simulink model "BlocoHidraulicoLAC_closeLoop"  (R2026a)
settings: Solver=ode15s  StopTime=5  FixedStep=0.001  MaxStep=1e-4
values from neighbouring files (symbols this model uses):
  Gamma = sys_d.B    [sintese_lqi_luenberger_lac.m]    (also in sintese_lqi_luenberger_lac_bateria_de_ensaio.m)
  K_i = -K_aug(3)    [sintese_lqi_luenberger_lac.m]    (also in sintese_lqi_luenberger_lac_bateria_de_ensaio.m)
  K_lqr = [K_pos, K_vel]    [sintese_lqi_luenberger_lac.m]    (also in sintese_lqi_luenberger_lac_bateria_de_ensaio.m)
  L_obs = place(Phi', Cx', polos_obs)'    [sintese_lqi_luenberger_lac.m]    (also in sintese_lqi_luenberger_lac_bateria_de_ensaio.m)
  Phi = sys_d.A    [sintese_lqi_luenberger_lac.m]    (also in sintese_lqi_luenberger_lac_bateria_de_ensaio.m)
undefined symbols (not defined in the file or in its folder): sigbuilder_block
(part 2 of 4)

== matlab function BlocoHidraulicoLAC_closeLoop/MATLAB Function ==
  settings: updateMethod=DISCRETE
  data: x_ref_mm input; duty_cycle_lac output; x_med_mm input; Phi input; Gamma input; K_lqr input; K_i input; L_obs input; dt input; x_est_mm output; v_est_mms output
function [duty_cycle_lac, x_est_mm, v_est_mms] = ...
    ecu_controle_posicao_lac_lqi(x_ref_mm, x_med_mm, Phi, Gamma, K_lqr, K_i, L_obs, dt)
%#codegen
% =========================================================================
% ECU AUTOMOTIVA: CONTROLE DE POSIÇÃO DO LAC VIA LQI + LUENBERGER
% Equivalente funcional do firmware em linguagem C (AURIX TC375)
% =========================================================================
% Entradas:
%   x_ref_mm       : Referência de deslocamento linear do êmbolo [mm]
%   x_med_mm       : Deslocamento medido pelo sensor/encoder da planta [mm]
%   Phi            : Matriz de estados do modelo discreto (2x2)
%   Gamma          : Vetor de entrada do modelo discreto (2x1)
%   K_lqr          : Ganhos dos estados proporcionais [K_pos, K_vel] (1x2)
%   K_i            : Ganho da ação integral de posição (escalar)
%   L_obs          : Vetor de ganhos do Observador de Luenberger (2x1)
%   dt             : Passo de amostragem numérico da ECU [s]
%
% Saídas:
%   duty_cycle_lac : Comando PWM de acionamento do motor [-100% a +100%]
%   x_est_mm       : Posição estimada pelo observador [mm]
%   v_est_mms      : Velocidade estimada pelo observador [mm/s]
% =========================================================================

%% 1. LIMITES MECÂNICOS DO ATUADOR FÍSICO
X_MIN_MM = 0.0;    % Batente mecânico traseiro (repouso) [mm]
X_MAX_MM = 53.7;   % Batente mecânico dianteiro (curso total) [mm]

%% 2. MEMÓRIA INTERNA DE ESTADOS (PERSISTENT / ESTÁTICAS DE FIRMWARE)
persistent xhat vhat integral_pos last_u
if isempty(xhat)
    xhat         = 0.0; % Posição estimada [mm]
    vhat         = 0.0; % Velocidade estimada [mm/s]
    integral_pos = 0.0; % Acumulador integral do erro [mm*s]
    last_u       = 0.0; % Último comando PWM efetivamente aplicado [-100 a +100]
end

%% 3. CONDICIONAMENTO DA REFERÊNCIA
% Garante que a referência nunca demande posição além dos fins de curso
x_ref_clamped = max(X_MIN_MM, min(X_MAX_MM, double(x_ref_mm)));
pos_real      = double(x_med_mm);

%% 4. OBSERVADOR DE LUENBERGER DISCRETO (PREDITOR-CORRETOR)
% Cálculo da inovação (erro de observação da saída de posição)
innov = pos_real - xhat;

% Atualização temporal dos estados estimados
xhat_new = Phi(1,1)*xhat + Phi(1,2)*vhat + Gamma(1)*last_u + L_obs(1)*innov;
vhat_new = Phi(2,1)*xhat + Phi(2,2)*vhat + Gamma(2)*last_u + L_obs(2)*innov;

xhat = xhat_new;
vhat = vhat_new;

%% 5. LEI DE CONTROLE LQI DE POSIÇÃO
erro_pos = x_ref_clamped - xhat;

% Candidato à integração do erro
integral_cand = integral_pos + erro_pos * dt;

% Lei de controle ótima não saturada
u_unclamped = (K_lqr(1) * erro_pos) - (K_lqr(2) * vhat) + (K_i * integral_cand);

%% 6. ANTI-WINDUP CONDICIONAL IDÊNTICO AO FIRMWARE AURIX
% Clamping rígido da ação integral quando satura na mesma direção do esforço
if (u_unclamped > 100.0 && erro_pos > 0.0)
    u_cmd = 100.0;
    % Congela a integração (não atualiza integral_pos)
elseif (u_unclamped < -100.0 && erro_pos < 0.0)
    u_cmd = -100.0;
    % Congela a integração (não atualiza integral_pos)
else
    integral_pos = integral_cand;
    u_cmd = u_unclamped;
    if u_cmd > 100.0
        u_cmd = 100.0;
    elseif u_cmd < -100.0
        u_cmd = -100.0;
    end
end

%% 7. ATUALIZAÇÃO DAS SAÍDAS E REGISTRADOR DE RETORNO
duty_cycle_lac = u_cmd;
last_u         = u_cmd;

x_est_mm  = xhat;
v_est_mms = vhat;

end
% function [duty_cycle_lac, u_mcv, u_pfv, u_irl, u_orl, x_est_mm, v_est_mms] = ...
%     ecu_controle_posicao_lac_lqi(x_ref_mm, x_med_mm, hab_adas, Phi, Gamma, K_lqr, K_i, L_obs, dt)
% %#codegen
% % =========================================================================
% % ECU AUTOMOTIVA: CONTROLE DE POSIÇÃO DO ATUADOR LINEAR (LAC) VIA LQI
% % =========================================================================
% % Entradas:
% %   x_ref_mm       : Posição de referência do êmbolo [mm]
% %   x_med_mm       : Posição medida pelo sensor/encoder da planta [mm]
% %   hab_adas       : Habilitação da função autônoma (1 = Ativo, 0 = Standby)
% %   Phi            : Matriz do modelo discreto (2x2) [pos; vel]
% %   Gamma          : Vetor de entrada do modelo discreto (2x1)
% %   K_lqr          : Vetor de ganhos dos estados [K_pos, K_vel] (1x2)
% %   K_i            : Ganho da ação integral de posição (escalar)
% %   L_obs          : Ganhos do Observador de Luenberger (2x1) [L_pos; L_vel]
% %   dt             : Período de amostragem do controle [s]
% %
% % Saídas:
% %   duty_cycle_lac : Sinal PWM para a ponte H do motor [-100% a +100%]
% %   u_mcv          : Válvula de corte mestre (NA: 1 = Energizada/Fechada)
% %   u_pfv          : Válvula de alimentação (NF: 1 = Energizada/Aberta)
% %   u_irl          : Válvula de entrada do caliper (NA: 0 = Aberta)
% %   u_orl          : Válvula de descarga/retorno (NF: 0 = Fechada)
% %   x_est_mm       : Posição estimada pelo observador [mm]
% %   v_est_mms      : Velocidade estimada pelo observador [mm/s]
% % =========================================================================
% 
% %% 1. LIMITES OPERACIONAIS E FÍSICOS
% X_MAX_MM = 53.7;  % Fim de curso mecânico máximo do êmbolo [mm]
% X_MIN_MM = 0.0;   % Posição de repouso mecânico do êmbolo [mm]
% 
% %% 2. MEMÓRIA INTERNA DE ESTADOS (PERSISTENT)
% persistent xhat vhat z_int u_ant
% if isempty(xhat)
%     xhat  = 0.0;  % Posição estimada [mm]
%     vhat  = 0.0;  % Velocidade estimada [mm/s]
%     z_int = 0.0;  % Integrador do erro de posição [mm*s]
%     u_ant = 0.0;  % Comando PWM anterior aplicado [-100 a +100]
% end
% 
% %% 3. CONDICIONAMENTO DAS ENTRADAS E REFERÊNCIAS
% % Saturação da referência de posição dentro dos batentes físicos
% x_ref_sat = max(X_MIN_MM, min(X_MAX_MM, double(x_ref_mm)));
% y_med     = double(x_med_mm);
% 
% %% 4. OBSERVADOR DE LUENBERGER DISCRETO (PREDITOR-CORRETOR)
% % Inovação baseada na leitura do sensor de posição físico
% innov = y_med - xhat;
% 
% % Predição e correção temporal de estados com as matrizes externas
% xhat_next = Phi(1,1)*xhat + Phi(1,2)*vhat + Gamma(1)*u_ant + L_obs(1)*innov;
% vhat_next = Phi(2,1)*xhat + Phi(2,2)*vhat + Gamma(2)*u_ant + L_obs(2)*innov;
% 
% % Atualização dos estados estimados
% xhat = xhat_next;
% vhat = vhat_next;
% 
% %% 5. GESTÃO OPERACIONAL DAS VÁLVULAS SOLENOIDES (MODO ADAS)
% if hab_adas > 0.5
%     % --- MODO ATIVO DE FRENAGEM (ACC / AEB) ---
%     % MCV fechada (isola pedal), PFV aberta (conecta LAC ao circuito)
%     % IRL aberta (livre fluxo para a pinça), ORL fechada (sem alívio ao dreno)
%     u_mcv = 1.0;
%     u_pfv = 1.0;
%     u_irl = 0.0; 
%     u_orl = 0.0;
% 
%     %% 6. LEI DE CONTROLE LQI DE POSIÇÃO
%     erro_pos = x_ref_sat - xhat;
% 
%     % Candidato à atualização integral
%     z_cand = z_int + erro_pos * dt;
% 
%     % Lei de controle LQI: u = -Kx*xhat + Ki*z
%     % u_lqi = K_lqr(1)*(x_ref - xhat) - K_lqr(2)*vhat + K_i*z
%     u_unclamped = (K_lqr(1) * erro_pos) - (K_lqr(2) * vhat) + (K_i * z_cand);
% 
%     % Saturação do atuador motor [-100% a +100%]
%     u_sat = max(-100.0, min(100.0, u_unclamped));
% 
%     % Anti-windup condicional por integração clamped
%     is_saturated = (u_sat ~= u_unclamped);
%     if is_saturated
%         % Congela o integrador se a saturação estiver na mesma direção do erro
%         if (u_sat >= 100.0 && erro_pos > 0.0) || (u_sat <= -100.0 && erro_pos < 0.0)
%             % Mantém z_int anterior (não integra)
%         else
%             z_int = z_cand;
%         end
%     else
%         z_int = z_cand;
%     end
% 
%     duty_cycle_lac = u_sat;
% 
% else
%     % --- MODO STANDBY / REPOUSO ---
%     % Circuito hidráulico despressurizado e conectado ao pedal/reservatório
%     u_mcv = 0.0; % Aberta
%     u_pfv = 0.0; % Fechada
%     u_irl = 0.0; % Aberta
%     u_orl = 0.0; % Fechada
% 
%     duty_cycle_lac = 0.0;
%     z_int = 0.0; % Zera integrador
% end
% 
% %% 7. ATUALIZAÇÃO DE REGISTRADORES E SAÍDAS DO BLOCO
% u_ant = duty_cycle_lac;
% 
% x_est_mm  = xhat;
% v_est_mms = vhat;
% 
% end
% 
% 
% 
% 
% % function [duty_cycle_ecu, u_mcv, u_pfv, u_irl, u_orl] = ecu_control_valves_fcn(P_roda_pa, P_ref_pa, K_est, K_i, L_obs, dt)
% % %#codegen
% % % =========================================================================
% % % ECU AUTOMOTIVA: CONTROLE INDIRETO DE PRESSÃO VIA POSIÇÃO DO LAC
% % % =========================================================================
% % % Entradas:
% % %   P_roda_pa  : Leitura do sensor de pressão no caliper [Pa]
% % %   P_ref_pa   : Referência de pressão enviada pelo piloto/sistema [Pa]
% % %   K_est      : Ganhos do LQI para estados [x, x_dot, P] (1x3)
% % %   K_i        : Ganho integral do LQI de posição (escalar)
% % %   L_obs      : Ganhos do Observador de Luenberger [L_vel; L_pres] (2x1)
% % %   dt         : Período de amostragem da ECU [s]
% % %
% % % Saídas:
% % %   duty_cycle_ecu : Comando PWM para a ponte H do motor [-100% a +100%]
% % %   u_mcv, u_pfv, u_irl, u_orl : Sinais ON/OFF para os solenoides das válvulas
% % % =========================================================================
% % 
% % %% 1. PARÂMETROS FIXOS DE MATRIZES DA ECU
% % A_lac   = 2.85e-4;       % Área do êmbolo do LAC [m^2]
% % tau_m   = 0.140;         % Constante de tempo mecânica [s]
% % K_drv   = 0.085;         % Ganho de velocidade fuso [m/s]
% % C_eq    = 9.51e-12;      % Capacitância equivalente [m^3/Pa]
% % 
% % % Submatrizes do observador reduzido de ordem 2 [x_dot; p]
% % A_sub = [-1.0/tau_m, 0.0;
% %           A_lac/C_eq, 0.0];
% % B_sub = [K_drv/tau_m; 
% %          0.0];
% % 
% % % Banda morta hidráulica de histerese (~1.5 PSI) para evitar oscilação de válvulas
% % BANDA_MORTA_PA = 1.5 * 6894.757;
% % 
% % %% 2. MEMÓRIA INTERNA DE ESTADOS ESTIMADOS DA ECU (PERSISTENT)
% % persistent x_est x_dot_est p_est erro_int_pos u_sat_ant
% % if isempty(x_est)
% %     x_est        = 0.0;
% %     x_dot_est    = 0.0;
% %     p_est        = 0.0;
% %     erro_int_pos = 0.0;
% %     u_sat_ant    = 0.0;
% % end
% % 
% % %% 3. MAPEAMENTO INDIRETO: PRESSÃO DE REFERÊNCIA -> POSIÇÃO DO LAC
% % % Em regime permanente hidráulico: delta_V = A_lac * x = C_eq * P
% % x_ref = (C_eq / A_lac) * double(P_ref_pa);
% % x_ref = max(0.0, min(0.0537, x_ref)); % Saturação no curso físico do atuador
% % 
% % %% 4. OBSERVADOR DE LUENBERGER REDUZIDO (ESTIMAÇÃO DE VELOCIDADE E PRESSÃO)
% % erro_estimacao = double(P_roda_pa) - p_est;
% % 
% % % Derivadas estimadas realimentadas pelo erro do sensor de pressão + comando anterior aplicado
% % x_dot_dot_est = A_sub(1,1)*x_dot_est + L_obs(1)*erro_estimacao + B_sub(1)*u_sat_ant;
% % p_dot_est     = A_sub(2,1)*x_dot_est + L_obs(2)*erro_estimacao;
% % 
% % % Integração numérica de Euler dos estados estimados
% % x_dot_est = x_dot_est + x_dot_dot_est * dt;
% % p_est     = max(0.0, p_est + p_dot_est * dt);
% % x_est     = max(0.0, min(0.0537, x_est + x_dot_est * dt));
% % 
% % %% 5. LEI DE CONTROLE LQI INDIRETO FOCADO NA POSIÇÃO DO LAC
% % % Erro instantâneo de deslocamento mecânico do fuso
% % erro_pos = x_ref - x_est;
% % 
% % % Cálculo da ação de controle ótimo por realimentação de estados + ação integral
% % % u = K_pos * (x_ref - x) - K_vel * x_dot + Ki * erro_integral
% % u_controle = K_est(1) * erro_pos - K_est(2) * x_dot_est + double(K_i) * erro_int_pos;
% % 
% % % Saturação física unitária do motor (-1.0 a +1.0)
% % u_sat = max(-1.0, min(1.0, u_controle));
% % 
% % %% 6. MÁQUINA DE ESTADOS HÍBRIDA (GERENCIAMENTO DAS VÁLVULAS)
% % erro_pressao_pa = double(P_ref_pa) - double(P_roda_pa);
% % 
% % if erro_pressao_pa > BANDA_MORTA_PA
% %     %% --- MODO APPLY (Aumento Ativo de Pressão) ---
% %     % Circuito conectado do LAC para a roda; dreno fechado
% %     u_mcv = 1; u_pfv = 1; u_irl = 1; u_orl = 0;
% % 
% %     % Acúmulo do integrador com Anti-Windup rígido no curso em metros
% %     erro_int_pos = erro_int_pos + erro_pos * dt;
% %     if erro_int_pos > 0.020;  erro_int_pos = 0.020;  end  % Máx: 20 mm.s
% %     if erro_int_pos < -0.020; erro_int_pos = -0.020; end
% % 
% %     duty_cycle_ecu = u_sat * 100.0;
% % 
% % elseif erro_pressao_pa < -BANDA_MORTA_PA
% %     %% --- MODO RELEASE (Alívio Rápido de Pressão) ---
% %     % Drena fluido do caliper para o reservatório
% %     u_mcv = 0; u_pfv = 0; u_irl = 0; u_orl = 1;
% % 
% %     % Reseta a ação integral para evitar overshoot no retorno
% %     erro_int_pos = 0.0;
% % 
% %     % Recuo seguro do LAC: acompanha x_ref de volta à posição inicial
% %     if x_est > 0.001
% %         duty_cycle_ecu = min(0.0, max(-50.0, u_sat * 100.0));
% %     else
% %         duty_cycle_ecu = 0.0;
% %     end
% % 
% % else
% %     %% --- MODO HOLD (Retenção Hidráulica no Patamar) ---
% %     % Válvulas calam o caliper retendo a pressão; desliga o motor para poupar energia
% %     u_mcv = 1; u_pfv = 0; u_irl = 0; u_orl = 0;
% % 
% %     duty_cycle_ecu = 0.0;
% % end
% % 
% % % Limitação final de segurança da ponte H
% % duty_cycle_ecu = max(-100.0, min(100.0, duty_cycle_ecu));
% % 
% % % Atualiza o comando efetivo repassado para o observador no próximo passo
% % u_sat_ant = duty_cycle_ecu / 100.0;
% % 
% % end
% % 
% % % function [duty_cycle_ecu, u_mcv, u_pfv, u_irl, u_orl] = ecu_control_valves_fcn(P_roda_pa, P_ref_pa, K_est, K_i, L_obs, dt)
% % % %#codegen
% % % % =========================================================================
% % % % ECU AUTOMOTIVA: CONTROLE INDIRETO DE PRESSÃO VIA POSIÇÃO DO LAC
% % % % =========================================================================
% % % % Entradas:
% % % %   P_roda_pa  : Leitura do sensor de pressão no caliper [Pa]
% % % %   P_ref_pa   : Referência de pressão enviada pelo piloto/sistema [Pa]
% % % %   K_est      : Ganhos do LQI para estados [x, x_dot, P] (1x3)
% % % %   K_i        : Ganho integral do LQI de posição (escalar)
% % % %   L_obs      : Ganhos do Observador de Luenberger [L_vel; L_pres] (2x1)
% % % %   dt         : Período de amostragem da ECU [s]
% % % %
% % % % Saídas:
% % % %   duty_cycle_ecu : Comando PWM para a ponte H do motor [-100% a +100%]
% % % %   u_mcv, u_pfv, u_irl, u_orl : Sinais ON/OFF para os solenoides das válvulas
% % % % =========================================================================
% % % 
% % % %% 1. PARÂMETROS FIXOS DE MATRIZES DA ECU
% % % A_lac   = 2.85e-4;       % Área do êmbolo do LAC [m^2]
% % % tau_m   = 0.140;         % Constante de tempo mecânica [s]
% % % K_drv   = 0.085;         % Ganho de velocidade fuso [m/s]
% % % C_eq    = 9.51e-12;      % Capacitância equivalente [m^3/Pa]
% % % 
% % % % Submatrizes do observador reduzido de ordem 2 [x_dot; p]
% % % A_sub = [-1.0/tau_m, 0.0;
% % %           A_lac/C_eq, 0.0];
% % % B_sub = [K_drv/tau_m; 
% % %          0.0];
% % % 
% % % % Banda morta hidráulica de histerese (~1.5 PSI) para evitar oscilação de válvulas
% % % BANDA_MORTA_PA = 1.5 * 6894.757;
% % % 
% % % %% 2. MEMÓRIA INTERNA DE ESTADOS ESTIMADOS DA ECU (PERSISTENT)
% % % persistent x_est x_dot_est p_est erro_int_pos
% % % if isempty(x_est)
% % %     x_est        = 0.0;
% % %     x_dot_est    = 0.0;
% % %     p_est        = 0.0;
% % %     erro_int_pos = 0.0;
% % % end
% % % 
% % % %% 3. MAPEAMENTO INDIRETO: PRESSÃO DE REFERÊNCIA -> POSIÇÃO DO LAC
% % % % Em regime permanente hidráulico: delta_V = A_lac * x = C_eq * P
% % % % Logo, a referência de curso mecânico do LAC é dada por:
% % % x_ref = (C_eq / A_lac) * double(P_ref_pa);
% % % x_ref = max(0.0, min(0.0537, x_ref)); % Saturação no curso físico do atuador
% % % 
% % % %% 4. OBSERVADOR DE LUENBERGER REDUZIDO (ESTIMAÇÃO DE VELOCIDADE E PRESSÃO)
% % % erro_estimacao = double(P_roda_pa) - p_est;
% % % 
% % % % Derivadas estimadas realimentadas pelo erro do sensor de pressão
% % % x_dot_dot_est = A_sub(1,1)*x_dot_est + L_obs(1)*erro_estimacao;
% % % p_dot_est     = A_sub(2,1)*x_dot_est + L_obs(2)*erro_estimacao;
% % % 
% % % % Adição do termo do atuador anterior saturado
% % % % (Nota: B_sub(1) atua na aceleração do fuso)
% % % persistent u_sat_ant
% % % if isempty(u_sat_ant)
% % %     u_sat_ant = 0.0;
% % % end
% % % x_dot_dot_est = x_dot_dot_est + B_sub(1) * u_sat_ant;
% % % 
% % % % Integração numérica de Euler dos estados estimados
% % % x_dot_est = x_dot_est + x_dot_dot_est * dt;
% % % p_est     = max(0.0, p_est + p_dot_est * dt);
% % % x_est     = max(0.0, min(0.0537, x_est + x_dot_est * dt));
% % % 
% % % %% 5. LEI DE CONTROLE LQI INDIRETO FOCADO NA POSIÇÃO DO LAC
% % % % Erro instantâneo de deslocamento mecânico do fuso
% % % erro_pos = x_ref - x_est;
% % % 
% % % % Cálculo da ação de controle ótimo por realimentação de estados + ação integral
% % % % u = K_pos * (x_ref - x) - K_vel * x_dot + Ki * erro_integral
% % % u_controle = K_est(1) * erro_pos - K_est(2) * x_dot_est + double(K_i) * erro_int_pos;
% % % 
% % % % Saturação física unitária do motor (-1.0 a +1.0)
% % % u_sat = max(-1.0, min(1.0, u_controle));
% % % u_sat_ant = u_sat;
% % % 
% % % %% 6. MÁQUINA DE ESTADOS HÍBRIDA (GERENCIAMENTO DAS VÁLVULAS)
% % % erro_pressao_pa = double(P_ref_pa) - double(P_roda_pa);
% % % 
% % % if erro_pressao_pa > BANDA_MORTA_PA
% % %     %% --- MODO APPLY (Aumento Ativo de Pressão) ---
% % %     % Circuito conectado do LAC para a roda; dreno fechado
% % %     u_mcv = 1; u_pfv = 1; u_irl = 1; u_orl = 0;
% % % 
% % %     % Acúmulo do integrador com Anti-Windup rígido no curso em metros
% % %     erro_int_pos = erro_int_pos + erro_pos * dt;
% % %     if erro_int_pos > 0.020;  erro_int_pos = 0.020;  end  % Máx: 20 mm.s
% % %     if erro_int_pos < -0.020; erro_int_pos = -0.020; end
% % % 
% % %     duty_cycle_ecu = u_sat * 100.0;
% % % 
% % % elseif erro_pressao_pa < -BANDA_MORTA_PA
% % %     %% --- MODO RELEASE (Alívio Rápido de Pressão) ---
% % %     % Drena fluido do caliper para o reservatório
% % %     u_mcv = 0; u_pfv = 0; u_irl = 0; u_orl = 1;
% % % 
% % %     % Reseta a ação integral para evitar overshoot no retorno
% % %     erro_int_pos = 0.0;
% % % 
% % %     % Recuo seguro do LAC: acompanha x_ref de volta à posição inicial
% % %     if x_est > 0.001
% % %         duty_cycle_ecu = min(0.0, max(-50.0, u_sat * 100.0));
% % %     else
% % %         duty_cycle_ecu = 0.0;
% % %     end
% % % 
% % % else
% % %     %% --- MODO HOLD (Retenção Hidráulica no Patamar) ---
% % %     % Válvulas calam o caliper retendo a pressão; desliga o motor para poupar energia
% % %     u_mcv = 1; u_pfv = 0; u_irl = 0; u_orl = 0;
% % % 
% % %     duty_cycle_ecu = 0.0;
% % % end
% % % 
% % % % Limitação final de segurança da ponte H
% % % duty_cycle_ecu = max(-100.0, min(100.0, duty_cycle_ecu));
% % % 
% % % end
% % % % function [duty_cycle_ecu, u_mcv, u_pfv, u_irl, u_orl] = ecu_control_valves_fcn(P_roda_pa, P_ref_pa, K_est, K_i, L_obs, dt)
% % % % %#codegen
% % % % % =========================================================================
% % % % % ECU AUTOMOTIVA: CONTROLE DIRETO E ROBUSTO DE PRESSÃO VIA LAC
% % % % % =========================================================================
% % % % 
% % % % %% 1. PARÂMETROS DA ECU
% % % % A_lac   = 2.85e-4;       % Área do êmbolo [m^2]
% % % % tau_m   = 0.140;         % Constante de tempo mecânica [s]
% % % % K_drv   = 0.085;         % Ganho de velocidade do fuso [m/s]
% % % % C_eq    = 9.51e-12;      % Capacitância equivalente [m^3/Pa]
% % % % 
% % % % % Submatrizes do observador de velocidade e pressão
% % % % A_sub = [-1.0/tau_m, 0.0;
% % % %     A_lac/C_eq, 0.0];
% % % % B_sub = [K_drv/tau_m; 
% % % %     0.0];
% % % % 
% % % % %% 2. MEMÓRIA INTERNA PERSISTENTE
% % % % persistent x_est x_dot_est p_est erro_int_p u_sat_ant
% % % % if isempty(x_est)
% % % %     x_est        = 0.0;
% % % %     x_dot_est    = 0.0;
% % % %     p_est        = 0.0;
% % % %     erro_int_p   = 0.0;
% % % %     u_sat_ant    = 0.0;
% % % % end
% % % % 
% % % % %% 3. ESTIMADOR DE ESTADOS (LUENBERGER)
% % % % erro_obs = double(P_roda_pa) - p_est;
% % % % 
% % % % x_dot_dot_est = A_sub(1,1)*x_dot_est + B_sub(1)*u_sat_ant + L_obs(1)*erro_obs;
% % % % p_dot_est     = A_sub(2,1)*x_dot_est + L_obs(2)*erro_obs;
% % % % 
% % % % x_dot_est = x_dot_est + x_dot_dot_est * dt;
% % % % p_est     = max(0.0, p_est + p_dot_est * dt);
% % % % x_est     = max(0.0, min(0.0537, x_est + x_dot_est * dt));
% % % % 
% % % % %% 4. LEI DE CONTROLE EM MALHA FECHADA DE PRESSÃO
% % % % erro_p = double(P_ref_pa) - double(P_roda_pa);
% % % % 
% % % % % Ganho de conversão pressão -> deslocamento equivalente
% % % % Kp_eff = (C_eq / A_lac); 
% % % % 
% % % % % Acúmulo integral com Anti-Windup rígido
% % % % erro_int_p = erro_int_p + erro_p * dt;
% % % % MAX_INT = 5.0e6; % Limite para evitar saturação do integrador
% % % % erro_int_p = max(-MAX_INT, min(MAX_INT, erro_int_p));
% % % % 
% % % % % Ação de controle: Proporcional ao erro de pressão + Derivativo via velocidade + Integral de pressão
% % % % u_prop = K_est(1) * (Kp_eff * erro_p);
% % % % u_der  = -K_est(2) * x_dot_est;
% % % % u_int  = (K_i * Kp_eff) * erro_int_p;
% % % % 
% % % % u_controle = u_prop + u_der + u_int;
% % % % 
% % % % % Saturação unitária da ponte H
% % % % u_sat = max(-1.0, min(1.0, u_controle));
% % % % u_sat_ant = u_sat;
% % % % 
% % % % %% 5. GERENCIAMENTO DAS VÁLVULAS HIDRÁULICAS
% % % % PSI_TO_PA = 6894.757;
% % % % 
% % % % if P_ref_pa <= (0.5 * PSI_TO_PA)
% % % %     %% MODO REPOUSO / ALÍVIO TOTAL (0 PSI)
% % % %     % Abre dreno da roda e recolhe êmbolo
% % % %     u_mcv = 0; 
% % % %     u_pfv = 0; 
% % % %     u_irl = 0; 
% % % %     u_orl = 1;
% % % % 
% % % %     erro_int_p = 0.0; % Reset integrador
% % % %     if x_est > 0.0005
% % % %         duty_cycle_ecu = -40.0; % Retrai LAC suavemente até fim de curso traseiro
% % % %     else
% % % %         duty_cycle_ecu = 0.0;
% % % %     end
% % % % else
% % % %     %% MODO MODULAÇÃO ATIVA DE PRESSÃO (Aumento, Retenção e Alívio Parcial)
% % % %     % Circuito conectado direto LAC <-> Caliper da roda (sem vazamento para tanque)
% % % %     u_mcv = 0;  % Fechada: bloqueia fuga para o reservatório principal
% % % %     u_pfv = 1;  % Aberta: conecta LAC à galeria principal
% % % %     u_irl = 1;  % Aberta: conecta galeria principal ao caliper
% % % %     u_orl = 0;  % Fechada: bloqueia dreno para manter fluido no sistema
% % % % 
% % % %     duty_cycle_ecu = u_sat * 100.0;
% % % % end
% % % % 
% % % % % Limitação de saída de segurança
% % % % duty_cycle_ecu = max(-100.0, min(100.0, duty_cycle_ecu));
% % % % 
% % % % end
% % % % 
% % % % % function [duty_cycle_ecu, u_mcv, u_pfv, u_irl, u_orl] = ecu_control_valves_fcn(P_roda_pa, P_ref_pa, K_est, K_i, L_obs, dt)
% % % % % %#codegen
% % % % % % =========================================================================
% % % % % % ECU AUTOMOTIVA: CONTROLE INDIRETO DE PRESSÃO VIA POSIÇÃO DO LAC
% % % % % % =========================================================================
% % % % % % Entradas:
% % % % % %   P_roda_pa  : Leitura do sensor de pressão no caliper [Pa]
% % % % % %   P_ref_pa   : Referência de pressão enviada pelo piloto/sistema [Pa]
% % % % % %   K_est      : Ganhos do LQI para estados [x, x_dot, P] (1x3)
% % % % % %   K_i        : Ganho integral do LQI de posição (escalar)
% % % % % %   L_obs      : Ganhos do Observador de Luenberger [L_vel; L_pres] (2x1)
% % % % % %   dt         : Período de amostragem da ECU [s]
% % % % % %
% % % % % % Saídas:
% % % % % %   duty_cycle_ecu : Comando PWM para a ponte H do motor [-100% a +100%]
% % % % % %   u_mcv, u_pfv, u_irl, u_orl : Sinais ON/OFF para os solenoides das válvulas
% % % % % % =========================================================================
% % % % % 
% % % % % %% 1. PARÂMETROS FIXOS DE MATRIZES DA ECU
% % % % % A_lac   = 2.85e-4;       % Área do êmbolo do LAC [m^2]
% % % % % tau_m   = 0.140;         % Constante de tempo mecânica [s]
% % % % % K_drv   = 0.085;         % Ganho de velocidade fuso [m/s]
% % % % % C_eq    = 9.51e-12;      % Capacitância equivalente [m^3/Pa]
% % % % % 
% % % % % % Submatrizes do observador reduzido de ordem 2 [x_dot; p]
% % % % % A_sub = [-1.0/tau_m, 0.0;
% % % % %           A_lac/C_eq, 0.0];
% % % % % B_sub = [K_drv/tau_m; 
% % % % %          0.0];
% % % % % 
% % % % % % Banda morta hidráulica de histerese (~1.5 PSI) para evitar oscilação de válvulas
% % % % % BANDA_MORTA_PA = 1.5 * 6894.757;
% % % % % 
% % % % % %% 2. MEMÓRIA INTERNA DE ESTADOS ESTIMADOS DA ECU (PERSISTENT)
% % % % % persistent x_est x_dot_est p_est erro_int_pos
% % % % % if isempty(x_est)
% % % % %     x_est        = 0.0;
% % % % %     x_dot_est    = 0.0;
% % % % %     p_est        = 0.0;
% % % % %     erro_int_pos = 0.0;
% % % % % end
% % % % % 
% % % % % %% 3. MAPEAMENTO INDIRETO: PRESSÃO DE REFERÊNCIA -> POSIÇÃO DO LAC
% % % % % % Em regime permanente hidráulico: delta_V = A_lac * x = C_eq * P
% % % % % % Logo, a referência de curso mecânico do LAC é dada por:
% % % % % x_ref = (C_eq / A_lac) * double(P_ref_pa);
% % % % % x_ref = max(0.0, min(0.0537, x_ref)); % Saturação no curso físico do atuador
% % % % % 
% % % % % %% 4. OBSERVADOR DE LUENBERGER REDUZIDO (ESTIMAÇÃO DE VELOCIDADE E PRESSÃO)
% % % % % erro_estimacao = double(P_roda_pa) - p_est;
% % % % % 
% % % % % % Derivadas estimadas realimentadas pelo erro do sensor de pressão
% % % % % x_dot_dot_est = A_sub(1,1)*x_dot_est + L_obs(1)*erro_estimacao;
% % % % % p_dot_est     = A_sub(2,1)*x_dot_est + L_obs(2)*erro_estimacao;
% % % % % 
% % % % % % Adição do termo do atuador anterior saturado
% % % % % % (Nota: B_sub(1) atua na aceleração do fuso)
% % % % % persistent u_sat_ant
% % % % % if isempty(u_sat_ant)
% % % % %     u_sat_ant = 0.0;
% % % % % end
% % % % % x_dot_dot_est = x_dot_dot_est + B_sub(1) * u_sat_ant;
% % % % % 
% % % % % % Integração numérica de Euler dos estados estimados
% % % % % x_dot_est = x_dot_est + x_dot_dot_est * dt;
% % % % % p_est     = max(0.0, p_est + p_dot_est * dt);
% % % % % x_est     = max(0.0, min(0.0537, x_est + x_dot_est * dt));
% % % % % 
% % % % % %% 5. LEI DE CONTROLE LQI INDIRETO FOCADO NA POSIÇÃO DO LAC
% % % % % % Erro instantâneo de deslocamento mecânico do fuso
% % % % % erro_pos = x_ref - x_est;
% % % % % 
% % % % % % Cálculo da ação de controle ótimo por realimentação de estados + ação integral
% % % % % % u = K_pos * (x_ref - x) - K_vel * x_dot + Ki * erro_integral
% % % % % u_controle = K_est(1) * erro_pos - K_est(2) * x_dot_est + double(K_i) * erro_int_pos;
% % % % % 
% % % % % % Saturação física unitária do motor (-1.0 a +1.0)
% % % % % u_sat = max(-1.0, min(1.0, u_controle));
% % % % % u_sat_ant = u_sat;
% % % % % 
% % % % % %% 6. MÁQUINA DE ESTADOS HÍBRIDA (GERENCIAMENTO DAS VÁLVULAS)
% % % % % erro_pressao_pa = double(P_ref_pa) - double(P_roda_pa);
% % % % % 
% % % % % if erro_pressao_pa > BANDA_MORTA_PA
% % % % %     %% --- MODO APPLY (Aumento Ativo de Pressão) ---
% % % % %     % Circuito conectado do LAC para a roda; dreno fechado
% % % % %     u_mcv = 1; u_pfv = 1; u_irl = 1; u_orl = 0;
% % % % % 
% % % % %     % Acúmulo do integrador com Anti-Windup rígido no curso em metros
% % % % %     erro_int_pos = erro_int_pos + erro_pos * dt;
% % % % %     if erro_int_pos > 0.020;  erro_int_pos = 0.020;  end  % Máx: 20 mm.s
% % % % %     if erro_int_pos < -0.020; erro_int_pos = -0.020; end
% % % % % 
% % % % %     duty_cycle_ecu = u_sat * 100.0;
% % % % % 
% % % % % elseif erro_pressao_pa < -BANDA_MORTA_PA
% % % % %     %% --- MODO RELEASE (Alívio Rápido de Pressão) ---
% % % % %     % Drena fluido do caliper para o reservatório
% % % % %     u_mcv = 0; u_pfv = 0; u_irl = 0; u_orl = 1;
% % % % % 
% % % % %     % Reseta a ação integral para evitar overshoot no retorno
% % % % %     erro_int_pos = 0.0;
% % % % % 
% % % % %     % Recuo seguro do LAC: acompanha x_ref de volta à posição inicial
% % % % %     if x_est > 0.001
% % % % %         duty_cycle_ecu = min(0.0, max(-50.0, u_sat * 100.0));
% % % % %     else
% % % % %         duty_cycle_ecu = 0.0;
% % % % %     end
% % % % % 
% % % % % else
% % % % %     %% --- MODO HOLD (Retenção Hidráulica no Patamar) ---
% % % % %     % Válvulas calam o caliper retendo a pressão; desliga o motor para poupar energia
% % % % %     u_mcv = 1; u_pfv = 0; u_irl = 0; u_orl = 0;
% % % % % 
% % % % %     duty_cycle_ecu = 0.0;
% % % % % end
% % % % % 
% % % % % % Limitação final de segurança da ponte H
% % % % % duty_cycle_ecu = max(-100.0, min(100.0, duty_cycle_ecu));
% % % % % 
% % % % % end
% % % % % 
% % % % % % function [duty_cycle_ecu, u_mcv, u_pfv, u_irl, u_orl] = ecu_control_valves_fcn(P_roda_pa, P_ref_pa, K_v, K_p, K_i, L_obs_d, Phi, Gamma, dt)
% % % % % % %#codegen
% % % % % % % =========================================================================
% % % % % % % ECU AUTOMOTIVA INTEGRADA (LQI DIGITAL + LUENBERGER + GESTÃO DE VÁLVULAS)
% % % % % % % Entradas:
% % % % % % %   P_roda_pa : Pressão medida na roda [Pa]
% % % % % % %   P_ref_pa  : Referência de pressão [Pa]
% % % % % % %   K_v, K_p, K_i : Ganhos sintonizados pelo LQI
% % % % % % %   L_obs_d   : Vetor [2x1] com ganhos discretos do observador
% % % % % % %   Phi, Gamma: Matrizes discretas do sistema [v; P]
% % % % % % %   dt        : Passo de integração [s]
% % % % % % % =========================================================================
% % % % % % 
% % % % % % %% 1. CONSTANTES E CONFIGURAÇÕES DE OPERAÇÃO
% % % % % % BANDA_MORTA_PA = 1.5 * 6894.757; % Banda morta de chaveamento (1.5 PSI em Pa)
% % % % % % WINDUP_LIMIT   = 1.5e5;          % Limite anti-windup em Pascal*s
% % % % % % 
% % % % % % %% 2. MEMÓRIA PERSISTENTE DA ECU (Estados Internos)
% % % % % % persistent v_est p_est erro_int u_sat_ant
% % % % % % if isempty(v_est)
% % % % % %     v_est     = 0.0;
% % % % % %     p_est     = 0.0;
% % % % % %     erro_int  = 0.0;
% % % % % %     u_sat_ant = 0.0;
% % % % % % end
% % % % % % 
% % % % % % %% 3. OBSERVADOR DE LUENBERGER DISCRETO
% % % % % % % Inovação baseada na saída medida do sensor
% % % % % % erro_obs = double(P_roda_pa) - p_est;
% % % % % % 
% % % % % % % Atualização com correção de saída e dinâmica de malha fechada
% % % % % % v_est_next = Phi(1,1)*v_est + Phi(1,2)*p_est + Gamma(1)*u_sat_ant + L_obs_d(1)*erro_obs;
% % % % % % p_est_next = Phi(2,1)*v_est + Phi(2,2)*p_est + Gamma(2)*u_sat_ant + L_obs_d(2)*erro_obs;
% % % % % % 
% % % % % % v_est = v_est_next;
% % % % % % p_est = p_est_next;
% % % % % % 
% % % % % % %% 4. GERENCIADOR DE ESTADOS HÍBRIDO (VÁLVULAS + CONTROLE)
% % % % % % erro_pressao = double(P_ref_pa) - double(P_roda_pa);
% % % % % % 
% % % % % % if erro_pressao > BANDA_MORTA_PA
% % % % % %     %% --- FASE 1: APPLY (Aumento Ativo de Pressão) ---
% % % % % %     % MCV = 0: Isola a linha do reservatório (Impede fuga do fluido na simulação)
% % % % % %     % PFV = 1: Alimenta da câmara do LAC para a linha principal
% % % % % %     % IRL = 1: Permite entrada do fluido no caliper da roda
% % % % % %     % ORL = 0: Saída de exaustão fechada
% % % % % %     u_mcv = 0;
% % % % % %     u_pfv = 1;
% % % % % %     u_irl = 1;
% % % % % %     u_orl = 0;
% % % % % % 
% % % % % %     % Atualização do integrador com Anti-Windup
% % % % % %     erro_int = erro_int + erro_pressao * dt;
% % % % % %     if erro_int > WINDUP_LIMIT;  erro_int = WINDUP_LIMIT;  end
% % % % % %     if erro_int < -WINDUP_LIMIT; erro_int = -WINDUP_LIMIT; end
% % % % % % 
% % % % % %     % Lei de Controle LQI no Espaço de Erro
% % % % % %     u_raw = - (K_v * v_est) - (K_p * (p_est - double(P_ref_pa))) + (K_i * erro_int);
% % % % % % 
% % % % % % elseif erro_pressao < -BANDA_MORTA_PA
% % % % % %     %% --- FASE 2: RELEASE (Alívio de Pressão Controlado) ---
% % % % % %     if double(P_ref_pa) <= 100.0
% % % % % %         % Despressurização rápida para retorno a zero
% % % % % %         u_mcv = 0;
% % % % % %         u_pfv = 1;
% % % % % %         u_irl = 1;
% % % % % %         u_orl = 1; % Abre exaustão suplementar para tanque
% % % % % %         erro_int = 0.0;
% % % % % %         u_raw = -0.30; % Recuo seguro a 30%
% % % % % %     else
% % % % % %         % Alívio proporcional fechado (ex: 200 PSI -> 50 PSI)
% % % % % %         u_mcv = 0;
% % % % % %         u_pfv = 1;
% % % % % %         u_irl = 1;
% % % % % %         u_orl = 0;
% % % % % % 
% % % % % %         erro_int = erro_int + erro_pressao * dt;
% % % % % %         if erro_int > WINDUP_LIMIT;  erro_int = WINDUP_LIMIT;  end
% % % % % %         if erro_int < -WINDUP_LIMIT; erro_int = -WINDUP_LIMIT; end
% % % % % % 
% % % % % %         u_raw = - (K_v * v_est) - (K_p * (p_est - double(P_ref_pa))) + (K_i * erro_int);
% % % % % %     end
% % % % % % 
% % % % % % else
% % % % % %     %% --- FASE 3: HOLD (Retenção Hidráulica em Patamar Estável) ---
% % % % % %     % Sela a pressão dentro do caliper da roda e desliga o motor elétrico
% % % % % %     u_mcv = 0;
% % % % % %     u_pfv = 1;
% % % % % %     u_irl = 0; % Sela o caliper mecanicamente
% % % % % %     u_orl = 0;
% % % % % % 
% % % % % %     u_raw = 0.0; % Desliga o esforço do motor para poupar energia
% % % % % %     % Congela erro_int sem acumular (anti-windup por parada de integração)
% % % % % % end
% % % % % % 
% % % % % % %% 5. SATURAÇÃO FÍSICA DO COMANDO
% % % % % % if u_raw > 1.0
% % % % % %     u_sat = 1.0;
% % % % % % elseif u_raw < -1.0
% % % % % %     u_sat = -1.0;
% % % % % % else
% % % % % %     u_sat = u_raw;
% % % % % % end
% % % % % % 
% % % % % % % Salva para o próximo passo do observador (elimina saturação descontrolada)
% % % % % % u_sat_ant = u_sat;
% % % % % % 
% % % % % % % Converte escala normalizada [-1.0, 1.0] para porcentagem [-100.0, 100.0]
% % % % % % duty_cycle_ecu = u_sat * 100.0;
% % % % % % 
% % % % % % end
% % % % % % 
% % % % % % % function [duty_cycle_ecu, u_mcv, u_pfv, u_irl, u_orl] = ecu_control_valves_fcn(P_roda_pa, P_ref_pa, K_est, K_i, L_obs, dt)
% % % % % % % %#codegen
% % % % % % % % ECU AUTOMOTIVA CONSOLIDADA - 100% SISTEMA INTERNACIONAL (PASCAL)
% % % % % % % % Inputs: 
% % % % % % % %   P_roda_pa : Pressão vinda da planta em Pascal [Pa]
% % % % % % % %   P_ref_pa  : Referência vinda do Script Mestre em Pascal [Pa]
% % % % % % % 
% % % % % % % %% 1. PARÂMETROS FIXOS DE MATRIZES DA ECU (Mesmos da Planta)
% % % % % % % A_lac   = 2.85e-4;   
% % % % % % % tau_m   = 0.140;   
% % % % % % % K_drv   = 0.085;   
% % % % % % % C_eq    = 9.51e-12;
% % % % % % % 
% % % % % % % % Matrizes do Sub-sistema de Ordem 2 (Velocidade e Pressão)
% % % % % % % A_sub = [-1/tau_m, 0;
% % % % % % %     A_lac/C_eq, 0];
% % % % % % % B_sub = [K_drv/tau_m; 0];
% % % % % % % 
% % % % % % % % Banda morta convertida para Pascal (~1.5 PSI)
% % % % % % % BANDA_MORTA_PA = 1.5 * 6894.757;
% % % % % % % 
% % % % % % % %% 2. MEMÓRIA INTERNA DE ESTADOS (PERSISTENT)
% % % % % % % persistent x_est x_dot_est p_est erro_int_acum
% % % % % % % if isempty(x_est)
% % % % % % %     x_est         = 0.0;
% % % % % % %     x_dot_est     = 0.0;
% % % % % % %     p_est         = 0.0;
% % % % % % %     erro_int_acum = 0.0;             
% % % % % % % end
% % % % % % % 
% % % % % % % %% 3. LEI DE CONTROLE LQI (Estrutura Canônica Clássica)
% % % % % % % z_vetor_est = [x_est; x_dot_est; p_est];
% % % % % % % 
% % % % % % % % Proteção de dimensão para garantir que K_est seja lido como vetor linha (1x3)
% % % % % % % K_row = reshape(K_est, 1, 3); 
% % % % % % % 
% % % % % % % % u = -K*z - Ki*integral_erro (Estrutura estável)
% % % % % % % u_controle = - (K_row * z_vetor_est) - (double(K_i) * erro_int_acum); 
% % % % % % % 
% % % % % % % % Saturação do atuador em escala unitária (-1.0 a 1.0) para o fuso
% % % % % % % u_sat = u_controle;
% % % % % % % if u_sat > 1.0;   u_sat = 1.0;   end
% % % % % % % if u_sat < -1.0;  u_sat = -1.0;  end
% % % % % % % 
% % % % % % % % Saída em escala de porcentagem (-100 a 100) exigida pela entrada da sua planta
% % % % % % % duty_cycle_ecu = u_sat * 100;
% % % % % % % 
% % % % % % % %% 4. OBSERVADOR DE LUENBERGER REDUZIDO (Ordem 2)
% % % % % % % % Alinhado com u_sat para evitar a explosão numérica que ocorria antes
% % % % % % % erro_estimacao = double(P_roda_pa) - p_est;
% % % % % % % 
% % % % % % % x_dot_dot_est  = A_sub(1,1)*x_dot_est + B_sub(1)*u_sat + L_obs(1)*erro_estimacao;
% % % % % % % p_dot_est      = A_sub(2,1)*x_dot_est + L_obs(2)*erro_estimacao;
% % % % % % % 
% % % % % % % % Integração numérica de Euler dos estados estimados
% % % % % % % x_dot_est = x_dot_est + x_dot_dot_est * dt;
% % % % % % % p_est     = p_est + p_dot_est * dt;
% % % % % % % x_est     = x_est + x_dot_est * dt;
% % % % % % % 
% % % % % % % %% 5. MÁQUINA DE ESTADOS HÍBRIDA (Chaveamento Dinâmico de Válvulas)
% % % % % % % erro_pa = double(P_ref_pa) - double(P_roda_pa);
% % % % % % % 
% % % % % % % if erro_pa > BANDA_MORTA_PA
% % % % % % %     %% --- MODO APPLY (Aumento) ---
% % % % % % %     u_mcv = 1; u_pfv = 1; u_irl = 1; u_orl = 0;
% % % % % % % 
% % % % % % %     % Integra o erro em Pascal
% % % % % % %     erro_int_acum = erro_int_acum + erro_pa * dt;
% % % % % % %     % Anti-Windup robusto em escala de Pascal
% % % % % % %     if erro_int_acum > 1e5;  erro_int_acum = 1e5;  end
% % % % % % %     if erro_int_acum < -1e5; erro_int_acum = -1e5; end
% % % % % % % 
% % % % % % % elseif erro_pa < -BANDA_MORTA_PA
% % % % % % %     %% --- MODO RELEASE (Alívio) ---
% % % % % % %     u_mcv = 0; u_pfv = 0; u_irl = 0; u_orl = 1;
% % % % % % % 
% % % % % % %     erro_int_acum  = 0.0; % Reseta a memória de força para evitar picos
% % % % % % %     duty_cycle_ecu = -30.0; % Recuo forçado seguro em malha aberta no alívio
% % % % % % % 
% % % % % % % else
% % % % % % %     %% --- MODO HOLD (Retenção) ---
% % % % % % %     u_mcv = 1; u_pfv = 0; u_irl = 0; u_orl = 0;
% % % % % % % 
% % % % % % %     % Como as válvulas travam o óleo, podemos desligar o motor para poupar energia
% % % % % % %     duty_cycle_ecu = 0.0; 
% % % % % % % end
% % % % % % % 
% % % % % % % end
% % % % % % % 
% % % % % % % % function [duty_cycle_ecu, u_mcv, u_pfv, u_irl, u_orl] = ecu_control_valves_fcn(P_roda_psi, P_ref_psi, K_est, K_i, L_obs, dt)
% % % % % % % % %#codegen
% % % % % % % % % ECU AUTOMOTIVA CONSOLIDADA: CORREÇÃO DE SATURAÇÃO DO OBSERVADOR
% % % % % % % % 
% % % % % % % % %% 1. PARÂMETROS E CONSTANTES
% % % % % % % % PSI_TO_PA = 6894.757;
% % % % % % % % A_lac = 2.85e-4;   tau_m = 0.140;   K_drv = 0.085;   C_eq = 9.51e-12;
% % % % % % % % 
% % % % % % % % A_sub = [-1/tau_m, 0; A_lac/C_eq, 0];
% % % % % % % % B_sub = [K_drv/tau_m; 0];
% % % % % % % % BANDA_MORTA_PSI = 1.5;
% % % % % % % % 
% % % % % % % % %% 2. MEMÓRIA INTERNA DE ESTADOS
% % % % % % % % persistent x_est x_dot_est p_est erro_int_acum
% % % % % % % % if isempty(x_est)
% % % % % % % %     x_est         = 0.0;
% % % % % % % %     x_dot_est     = 0.0;
% % % % % % % %     p_est         = 0.0;
% % % % % % % %     erro_int_acum = 0.0;             
% % % % % % % % end
% % % % % % % % 
% % % % % % % % %% 3. LEITURA DOS SENSORES E CONVERSÃO
% % % % % % % % P_roda_pa = double(P_roda_psi) * PSI_TO_PA;
% % % % % % % % P_ref_pa  = double(P_ref_psi) * PSI_TO_PA;
% % % % % % % % erro_psi  = double(P_ref_psi) - double(P_roda_psi);
% % % % % % % % 
% % % % % % % % %% 4. LEI DE CONTROLE LQI (Cálculo do sinal bruto)
% % % % % % % % z_vetor_est = [x_est; x_dot_est; p_est];
% % % % % % % % K_row = reshape(K_est, 1, 3); 
% % % % % % % % 
% % % % % % % % % Equação canônica do LQI do MATLAB
% % % % % % % % u_bruto = - (K_row * z_vetor_est) - (double(K_i) * erro_int_acum); 
% % % % % % % % 
% % % % % % % % % --- CORREÇÃO DE ENGENHARIA CRÍTICA: SATURAÇÃO DO ATUADOR ---
% % % % % % % % % Limita o sinal de controle físico entre -1.0 e 1.0 (escala do K_drv)
% % % % % % % % u_sat = u_bruto;
% % % % % % % % if u_sat > 1.0;   u_sat = 1.0;   end
% % % % % % % % if u_sat < -1.0;  u_sat = -1.0;  end
% % % % % % % % 
% % % % % % % % % O motor recebe o sinal saturado em escala de porcentagem (-100 a 100%)
% % % % % % % % duty_cycle_ecu = u_sat * 100;
% % % % % % % % 
% % % % % % % % %% 5. OBSERVADOR DE LUENBERGER REDUZIDO (Alimentado com u_sat correto!)
% % % % % % % % erro_estimacao = P_roda_pa - p_est;
% % % % % % % % 
% % % % % % % % % Usando u_sat (limitado) em vez de u_bruto para impedir a explosão numérica!
% % % % % % % % x_dot_dot_est  = A_sub(1,1)*x_dot_est + B_sub(1)*u_sat + L_obs(1)*erro_estimacao;
% % % % % % % % p_dot_est      = A_sub(2,1)*x_dot_est + L_obs(2)*erro_estimacao;
% % % % % % % % 
% % % % % % % % x_dot_est = x_dot_est + x_dot_dot_est * dt;
% % % % % % % % p_est     = p_est + p_dot_est * dt;
% % % % % % % % x_est     = x_est + x_dot_est * dt;
% % % % % % % % 
% % % % % % % % %% 6. MÁQUINA DE ESTADOS HÍBRIDA (GERENCIAMENTO REAL DE FLUXO)
% % % % % % % % 
% % % % % % % % % O integrador do LQI deve calcular continuamente o erro em todas as fases 
% % % % % % % % % para que o Observador não perca o rastreamento do fuso mecânico!
% % % % % % % % erro_int_acum = erro_int_acum + (P_ref_pa - P_roda_pa) * dt;
% % % % % % % % 
% % % % % % % % % Anti-Windup global unificado para proteger a saturação
% % % % % % % % if erro_int_acum > 1e5;  erro_int_acum = 1e5;  end
% % % % % % % % if erro_int_acum < -1e5; erro_int_acum = -1e5; end
% % % % % % % % 
% % % % % % % % % Cálculo contínuo do esforço do motor
% % % % % % % % duty_cycle_ecu = u_controle * 100;
% % % % % % % % 
% % % % % % % % if erro_psi > BANDA_MORTA_PSI
% % % % % % % %     %% --- MODO APPLY (Aumento Ativo) ---
% % % % % % % %     u_mcv = 1; u_pfv = 1; u_irl = 1; u_orl = 0;
% % % % % % % % 
% % % % % % % % elseif erro_psi < -BANDA_MORTA_PSI
% % % % % % % %     %% --- MODO RELEASE (Alívio Ativo) ---
% % % % % % % %     u_mcv = 0; u_pfv = 0; u_irl = 0; u_orl = 1;
% % % % % % % % 
% % % % % % % %     % Em vez de travar o motor em -30 fixo, deixa o LQI calcular 
% % % % % % % %     % o recuo controlado ideal baseado no erro negativo!
% % % % % % % % 
% % % % % % % % else
% % % % % % % %     %% --- MODO HOLD (Retenção Hidráulica) ---
% % % % % % % %     u_mcv = 1; u_pfv = 0; u_irl = 0; u_orl = 0;
% % % % % % % % 
% % % % % % % %     % Válvulas fechadas isolam o óleo, zeramos o PWM para poupar o motor
% % % % % % % %     duty_cycle_ecu = 0.0; 
% % % % % % % % end
% % % % % % % % 
% % % % % % % % % %% 6. MÁQUINA DE ESTADOS HÍBRIDA
% % % % % % % % % if erro_psi > BANDA_MORTA_PSI
% % % % % % % % %     %% --- MODO APPLY ---
% % % % % % % % %     u_mcv = 1; u_pfv = 1; u_irl = 1; u_orl = 0;
% % % % % % % % % 
% % % % % % % % %     % Acumula o erro e aplica proteção rígida contra estouro (Anti-Windup)
% % % % % % % % %     erro_int_acum = erro_int_acum + (P_ref_pa - P_roda_pa) * dt;
% % % % % % % % %     if erro_int_acum > 1e5;  erro_int_acum = 1e5;  end
% % % % % % % % %     if erro_int_acum < -1e5; erro_int_acum = -1e5; end
% % % % % % % % % 
% % % % % % % % % elseif erro_psi < -BANDA_MORTA_PSI
% % % % % % % % %     %% --- MODO RELEASE ---
% % % % % % % % %     u_mcv = 0; u_pfv = 0; u_irl = 0; u_orl = 1;
% % % % % % % % %     erro_int_acum  = 0.0; 
% % % % % % % % %     duty_cycle_ecu = -30.0; % Recuo forçado seguro
% % % % % % % % % 
% % % % % % % % % else
% % % % % % % % %     %% --- MODO HOLD ---
% % % % % % % % %     u_mcv = 1; u_pfv = 0; u_irl = 0; u_orl = 0;
% % % % % % % % %     % Mantém o motor ligado dosando o torque necessário para segurar a posição
% % % % % % % % % end
% % % % % % % % 
% % % % % % % % end
% % % % % % % % 
% % % % % % % % % function [duty_cycle_ecu, u_mcv, u_pfv, u_irl, u_orl] = ecu_control_valves_fcn(P_roda_psi, P_ref_psi, K_est, K_i, L_obs, dt)
% % % % % % % % % %#codegen
% % % % % % % % % % ECU AUTOMOTIVA INTEGRADA DINÂMICA
% % % % % % % % % % Agora os ganhos entram pelas portas K_est, K_i e L_obs vindos do script!
% % % % % % % % % 
% % % % % % % % % %% 1. REMOVIDOS OS NÚMEROS FIXOS. O bloco agora usa os parâmetros das portas.
% % % % % % % % % PSI_TO_PA = 6894.757;
% % % % % % % % % A_lac = 2.85e-4;   tau_m = 0.140;   K_drv = 0.085;   C_eq = 9.51e-12;
% % % % % % % % % 
% % % % % % % % % A_sub = [-1/tau_m, 0; A_lac/C_eq, 0];
% % % % % % % % % B_sub = [K_drv/tau_m; 0];
% % % % % % % % % BANDA_MORTA_PSI = 1.5;
% % % % % % % % % 
% % % % % % % % % %% 2. MEMÓRIA INTERNA DE ESTADOS
% % % % % % % % % persistent x_est x_dot_est p_est erro_int_acum
% % % % % % % % % if isempty(x_est)
% % % % % % % % %     x_est         = 0.0;
% % % % % % % % %     x_dot_est     = 0.0;
% % % % % % % % %     p_est         = 0.0;
% % % % % % % % %     erro_int_acum = 0.0;             
% % % % % % % % % end
% % % % % % % % % 
% % % % % % % % % %% 3. LEITURA DOS SENSORES E CONVERSÃO
% % % % % % % % % P_roda_pa = double(P_roda_psi) * PSI_TO_PA;
% % % % % % % % % P_ref_pa  = double(P_ref_psi) * PSI_TO_PA;
% % % % % % % % % erro_psi  = double(P_ref_psi) - double(P_roda_psi);
% % % % % % % % % 
% % % % % % % % % %% 4. LEI DE CONTROLE SINTONIZADA PELO LQI DO SCRIPT
% % % % % % % % % z_vetor_est = [x_est; x_dot_est; p_est];
% % % % % % % % % 
% % % % % % % % % % Force K_est to be a row vector by using the reshape or transpose operator (.')
% % % % % % % % % K_row = reshape(K_est, 1, 3); 
% % % % % % % % % 
% % % % % % % % % % u = -K*z - Ki*erro_acumulado
% % % % % % % % % u_controle  = - (K_row * z_vetor_est) - (double(K_i) * erro_int_acum); 
% % % % % % % % % % % Estrutura clássica de espaço de estados: u = -K*z - Ki*erro_acumulado
% % % % % % % % % % % Nota: Se o seu script gera o Ki positivo, mantemos o sinal de menos.
% % % % % % % % % % u_controle  = - (K_est * z_vetor_est) - (K_i * erro_int_acum); 
% % % % % % % % % % u_controle = - (K_est(1)*x_est + K_est(2)*x_dot_est + K_est(3)*p_est) - (double(K_i) * erro_int_acum);
% % % % % % % % % 
% % % % % % % % % 
% % % % % % % % % % Observador de Luenberger Reduzido (Usando L_obs dinâmico)
% % % % % % % % % erro_estimacao = P_roda_pa - p_est;
% % % % % % % % % x_dot_dot_est  = A_sub(1,1)*x_dot_est + B_sub(1)*u_controle + L_obs(1)*erro_estimacao;
% % % % % % % % % p_dot_est      = A_sub(2,1)*x_dot_est + L_obs(2)*erro_estimacao;
% % % % % % % % % 
% % % % % % % % % x_dot_est = x_dot_est + x_dot_dot_est * dt;
% % % % % % % % % p_est     = p_est + p_dot_est * dt;
% % % % % % % % % x_est     = x_est + x_dot_est * dt;
% % % % % % % % % 
% % % % % % % % % %% 5. MÁQUINA DE ESTADOS HÍBRIDA
% % % % % % % % % if erro_psi > BANDA_MORTA_PSI
% % % % % % % % %     u_mcv = 1; u_pfv = 1; u_irl = 1; u_orl = 0;
% % % % % % % % %     erro_int_acum = erro_int_acum + (P_ref_pa - P_roda_pa) * dt;
% % % % % % % % %     % Anti-Windup escalonado em Pascal para evitar o congelamento
% % % % % % % % %     if erro_int_acum > 1e6;  erro_int_acum = 1e6;  end
% % % % % % % % %     if erro_int_acum < -1e6; erro_int_acum = -1e6; end
% % % % % % % % %     duty_cycle_ecu = u_controle * 100;
% % % % % % % % % elseif erro_psi < -BANDA_MORTA_PSI
% % % % % % % % %     u_mcv = 0; u_pfv = 0; u_irl = 0; u_orl = 1;
% % % % % % % % %     erro_int_acum  = 0.0; 
% % % % % % % % %     duty_cycle_ecu = -30.0; 
% % % % % % % % % else
% % % % % % % % %     u_mcv = 1; u_pfv = 0; u_irl = 0; u_orl = 0;
% % % % % % % % %     duty_cycle_ecu = u_controle * 100; 
% % % % % % % % % end
% % % % % % % % % 
% % % % % % % % % %% 6. SATURAÇÃO
% % % % % % % % % if duty_cycle_ecu > 100.0;   duty_cycle_ecu = 100.0;   end
% % % % % % % % % if duty_cycle_ecu < -100.0;  duty_cycle_ecu = -100.0;  end
% % % % % % % % % 
% % % % % % % % % end
% % % % % % % % % 
% % % % % % % % % % function [duty_cycle_ecu, u_mcv, u_pfv, u_irl, u_orl] = ecu_control_valves_fcn(P_roda_psi, P_ref_psi, dt)
% % % % % % % % % % %#codegen
% % % % % % % % % % % ECU REVISADA: LQI + OBSERVADOR REDUZIDO + CONTROLE DE MCV E ALÍVIO PARCIAL
% % % % % % % % % % 
% % % % % % % % % % %% 1. GANHOS DO CONTROLADOR (Sintonizados para amortecer o choque inicial)
% % % % % % % % % % K_est = [15.54,   0.124,   0.00045];  
% % % % % % % % % % K_i   = -0.0065;                        
% % % % % % % % % % L_obs = [2250.5;  85.4]; 
% % % % % % % % % % 
% % % % % % % % % % % Constantes Físicas
% % % % % % % % % % PSI_TO_PA = 6894.757;
% % % % % % % % % % A_lac = 2.85e-4;   tau_m = 0.140;   K_drv = 0.085;   C_eq = 9.51e-12;
% % % % % % % % % % 
% % % % % % % % % % A_sub = [-1/tau_m, 0; A_lac/C_eq, 0];
% % % % % % % % % % B_sub = [K_drv/tau_m; 0];
% % % % % % % % % % 
% % % % % % % % % % BANDA_MORTA_PSI = 1.5;
% % % % % % % % % % 
% % % % % % % % % % %% 2. MEMÓRIA INTERNA DE ESTADOS
% % % % % % % % % % persistent x_est x_dot_est p_est erro_int_acum
% % % % % % % % % % if isempty(x_est)
% % % % % % % % % %     x_est         = 0.0;
% % % % % % % % % %     x_dot_est     = 0.0;
% % % % % % % % % %     p_est         = 0.0;
% % % % % % % % % %     erro_int_acum = 0.0;             
% % % % % % % % % % end
% % % % % % % % % % 
% % % % % % % % % % %% 3. LEITURA DOS SENSORES E CONVERSÃO
% % % % % % % % % % P_roda_pa = double(P_roda_psi) * PSI_TO_PA;
% % % % % % % % % % P_ref_pa  = double(P_ref_psi) * PSI_TO_PA;
% % % % % % % % % % erro_psi  = double(P_ref_psi) - double(P_roda_psi);
% % % % % % % % % % 
% % % % % % % % % % %% 4. LEI DE CONTROLE E OBSERVADOR DE LUENBERGER
% % % % % % % % % % z_vetor_est = [x_est; x_dot_est; p_est];
% % % % % % % % % % u_controle  = - (K_est * z_vetor_est) + (K_i * erro_int_acum);
% % % % % % % % % % 
% % % % % % % % % % erro_estimacao = P_roda_pa - p_est;
% % % % % % % % % % x_dot_dot_est  = A_sub(1,1)*x_dot_est + B_sub(1)*u_controle + L_obs(1)*erro_estimacao;
% % % % % % % % % % p_dot_est      = A_sub(2,1)*x_dot_est + L_obs(2)*erro_estimacao;
% % % % % % % % % % 
% % % % % % % % % % x_dot_est = x_dot_est + x_dot_dot_est * dt;
% % % % % % % % % % p_est     = p_est + p_dot_est * dt;
% % % % % % % % % % x_est     = x_est + x_dot_est * dt;
% % % % % % % % % % 
% % % % % % % % % % %% 5. MAQUINA DE ESTADOS HÍBRIDA (GERENCIADOR DE VÁLVULAS AUTOMOTIVAS)
% % % % % % % % % % 
% % % % % % % % % % if erro_psi > BANDA_MORTA_PSI
% % % % % % % % % %     %% --- MODO APPLY (Aumento de Pressão) ---
% % % % % % % % % %     u_mcv = 1; % FECHA a MCV (bloqueia o retorno ao reservatório)
% % % % % % % % % %     u_pfv = 1; % Abre alimentação do LAC
% % % % % % % % % %     u_irl = 1; % Abre entrada da roda
% % % % % % % % % %     u_orl = 0; % Fecha exaustão
% % % % % % % % % % 
% % % % % % % % % %     % Integração com Anti-Windup dinâmico rígido
% % % % % % % % % %     erro_int_acum = erro_int_acum + (P_ref_pa - P_roda_pa) * dt;
% % % % % % % % % %     if erro_int_acum > 2500.0;  erro_int_acum = 2500.0;  end
% % % % % % % % % %     if erro_int_acum < -2500.0; erro_int_acum = -2500.0; end
% % % % % % % % % % 
% % % % % % % % % %     duty_cycle_ecu = u_controle * 100;
% % % % % % % % % % 
% % % % % % % % % % elseif erro_psi < -BANDA_MORTA_PSI
% % % % % % % % % %     %% --- MODO RELEASE / DUMP (Alívio Parcial ou Total) ---
% % % % % % % % % %     u_mcv = 0; % Abre MCV para aliviar a linha principal
% % % % % % % % % %     u_pfv = 0; 
% % % % % % % % % %     u_irl = 0; % Isola o LAC
% % % % % % % % % %     u_orl = 1; % ABRE A DESCARGA: Libera óleo da roda para o reservatório cair a pressão
% % % % % % % % % % 
% % % % % % % % % %     erro_int_acum  = 0.0; % Reseta integrador para evitar rampa fantasma
% % % % % % % % % %     duty_cycle_ecu = -25.0; % Motor recua suavemente para abrir espaço na câmara
% % % % % % % % % % 
% % % % % % % % % % else
% % % % % % % % % %     %% --- MODO HOLD (Retenção e Estabilização no Patamar) ---
% % % % % % % % % %     u_mcv = 1; % Mantém fechada para preservar o circuito isolado
% % % % % % % % % %     u_pfv = 0; 
% % % % % % % % % %     u_irl = 0; % FECHA A IRL: Sela hidraulicamente o óleo estável dentro do caliper
% % % % % % % % % %     u_orl = 0; 
% % % % % % % % % % 
% % % % % % % % % %     duty_cycle_ecu = 0.0; % Desliga o motor elétrico (fuso segura a carga)
% % % % % % % % % % end
% % % % % % % % % % 
% % % % % % % % % % %% 6. SATURAÇÃO DA SAÍDA DA PONTE H
% % % % % % % % % % if duty_cycle_ecu > 100.0;   duty_cycle_ecu = 100.0;   end
% % % % % % % % % % if duty_cycle_ecu < -100.0;  duty_cycle_ecu = -100.0;  end
% % % % % % % % % % 
% % % % % % % % % % end
% % % % % % % % % % % function [duty_cycle_ecu, u_mcv, u_pfv, u_irl, u_orl] = ecu_control_valves_fcn(P_roda_psi, P_ref_psi, dt)
% % % % % % % % % % % %#codegen
% % % % % % % % % % % % ECU AUTOMOTIVA FIXADA: LQI + OBSERVADOR REDUZIDO + CHAVEAMENTO DE VÁLVULAS
% % % % % % % % % % % 
% % % % % % % % % % % %% 1. GANHOS DO CONTROLADOR (Substitua pelos valores gerados pelo script acima)
% % % % % % % % % % % K_est = [3.1623,   0.0242,   0.000302];  
% % % % % % % % % % % K_i   = -22.3607;                        
% % % % % % % % % % % L_obs = [1654.21;  42.85]; % Ganho do observador de ordem 2 [L1; L2]             
% % % % % % % % % % % 
% % % % % % % % % % % % Constantes Físicas de Conversão da ECU
% % % % % % % % % % % PSI_TO_PA = 6894.757;
% % % % % % % % % % % A_lac     = 2.85e-4;   
% % % % % % % % % % % tau_m     = 0.140;   
% % % % % % % % % % % K_drv     = 0.085;   
% % % % % % % % % % % C_eq      = 9.51e-12;
% % % % % % % % % % % 
% % % % % % % % % % % % Matrizes do Sub-sistema de Estimação de Ordem 2 (Velocidade e Pressão)
% % % % % % % % % % % A_sub = [-1/tau_m, 0;
% % % % % % % % % % %     A_lac/C_eq, 0];
% % % % % % % % % % % B_sub = [K_drv/tau_m; 0];
% % % % % % % % % % % 
% % % % % % % % % % % BANDA_MORTA_PSI = 2.0;
% % % % % % % % % % % 
% % % % % % % % % % % %% 2. MEMÓRIA INTERNA DE ESTADOS DA ECU
% % % % % % % % % % % persistent x_est x_dot_est p_est erro_int_acum
% % % % % % % % % % % if isempty(x_est)
% % % % % % % % % % %     x_est         = 0.0;
% % % % % % % % % % %     x_dot_est     = 0.0;
% % % % % % % % % % %     p_est         = 0.0;
% % % % % % % % % % %     erro_int_acum = 0.0;             
% % % % % % % % % % % end
% % % % % % % % % % % 
% % % % % % % % % % % %% 3. LEITURA DOS SENSORES
% % % % % % % % % % % P_roda_pa = double(P_roda_psi) * PSI_TO_PA;
% % % % % % % % % % % P_ref_pa  = double(P_ref_psi) * PSI_TO_PA;
% % % % % % % % % % % erro_psi  = double(P_ref_psi) - double(P_roda_psi);
% % % % % % % % % % % 
% % % % % % % % % % % %% 4. LEI DO CONTROLADOR INTEGRADO (Ação de Controle u)
% % % % % % % % % % % % Agrupa o vetor de estados estimado [x, x_dot, P] para a multiplicação do LQI
% % % % % % % % % % % z_vetor_est = [x_est; x_dot_est; p_est];
% % % % % % % % % % % u_controle  = - (K_est * z_vetor_est) + (K_i * erro_int_acum);
% % % % % % % % % % % 
% % % % % % % % % % % %% 5. ATUALIZAÇÃO DO OBSERVADOR DE ORDEM REDUZIDA (Via Integração de Euler)
% % % % % % % % % % % erro_estimacao = P_roda_pa - p_est;
% % % % % % % % % % % 
% % % % % % % % % % % % Derivadas do sub-sistema
% % % % % % % % % % % x_dot_dot_est = A_sub(1,1)*x_dot_est + B_sub(1)*u_controle + L_obs(1)*erro_estimacao;
% % % % % % % % % % % p_dot_est     = A_sub(2,1)*x_dot_est + L_obs(2)*erro_estimacao;
% % % % % % % % % % % 
% % % % % % % % % % % % Atualização dos estados estimados para o próximo milissegundo
% % % % % % % % % % % x_dot_est = x_dot_est + x_dot_dot_est * dt;
% % % % % % % % % % % p_est     = p_est + p_dot_est * dt;
% % % % % % % % % % % x_est     = x_est + x_dot_est * dt; % Posição integrada diretamente da velocidade
% % % % % % % % % % % 
% % % % % % % % % % % %% 6. GERENCIADOR LÓGICO DE FASE (APPLY, HOLD, RELEASE)
% % % % % % % % % % % 
% % % % % % % % % % % if erro_psi > BANDA_MORTA_PSI
% % % % % % % % % % %     %% --- MODO APPLY ---
% % % % % % % % % % %     u_mcv = 0; u_pfv = 1; u_irl = 1; u_orl = 0;
% % % % % % % % % % % 
% % % % % % % % % % %     erro_pressao  = P_ref_pa - P_roda_pa;
% % % % % % % % % % %     erro_int_acum = erro_int_acum + erro_pressao * dt;
% % % % % % % % % % %     duty_cycle_ecu = u_controle * 100;
% % % % % % % % % % % 
% % % % % % % % % % % elseif erro_psi < -BANDA_MORTA_PSI
% % % % % % % % % % %     %% --- MODO RELEASE ---
% % % % % % % % % % %     u_mcv = 0; u_pfv = 0; u_irl = 0; u_orl = 1;
% % % % % % % % % % % 
% % % % % % % % % % %     erro_int_acum  = 0.0; % Anti-windup
% % % % % % % % % % %     duty_cycle_ecu = -30.0; % Recuo seguro padrão de frenagem
% % % % % % % % % % % 
% % % % % % % % % % % else
% % % % % % % % % % %     %% --- MODO HOLD ---
% % % % % % % % % % %     u_mcv = 0; u_pfv = 0; u_irl = 0; u_orl = 0;
% % % % % % % % % % % 
% % % % % % % % % % %     duty_cycle_ecu = 0.0; % Desliga o motor elétrico (travamento mecânico hidráulico)
% % % % % % % % % % % end
% % % % % % % % % % % 
% % % % % % % % % % % %% 7. SATURAÇÃO DA PONTE H DA ECU
% % % % % % % % % % % if duty_cycle_ecu > 100.0
% % % % % % % % % % %     duty_cycle_ecu = 100.0;
% % % % % % % % % % % elseif duty_cycle_ecu < -100.0
% % % % % % % % % % %     duty_cycle_ecu = -100.0;
% % % % % % % % % % % end
% % % % % % % % % % % 
% % % % % % % % % % % end
% % % % % % % % % % % 
% % % % % % % % % % % % function [duty_cycle_ecu, u_mcv, u_pfv, u_irl, u_orl] = ecu_control_valves_fcn(P_roda_psi, P_ref_psi, dt)
% % % % % % % % % % % % %#codegen
% % % % % % % % % % % % % ECU AUTOMOTIVA CONSOLIDADA: LQI + OBSERVADOR + GERENCIADOR DE VÁLVULAS
% % % % % % % % % % % % % Sinais de Saída Digitais para os Relés/Transistores das Válvulas:
% % % % % % % % % % % % %   u_mcv, u_pfv, u_irl, u_orl : 0 (Fechada) ou 1 (Aberta)
% % % % % % % % % % % % 
% % % % % % % % % % % % %% 1. GANHOS DO CONTROLADOR (Idênticos ao cálculo anterior)
% % % % % % % % % % % % K_est = [3.1623,   0.0242,   0.000302];  
% % % % % % % % % % % % K_i   = -22.3607;                        
% % % % % % % % % % % % L     = [21.41; 1654.21; 42.85];             
% % % % % % % % % % % % 
% % % % % % % % % % % % % Constantes e Matrizes de Espaço de Estados da Planta
% % % % % % % % % % % % PSI_TO_PA = 6894.757;
% % % % % % % % % % % % A_lac     = 2.85e-4;   tau_m = 0.140;   K_drv = 0.085;   C_eq = 9.51e-12;
% % % % % % % % % % % % 
% % % % % % % % % % % % A = [0, 1, 0; 0, -1/tau_m, 0; 0, A_lac/C_eq, 0];
% % % % % % % % % % % % B = [0; K_drv/tau_m; 0];
% % % % % % % % % % % % C =0;
% % % % % % % % % % % % 
% % % % % % % % % % % % % Banda morta de pressão para evitar trepidação das válvulas (ex: 2.0 PSI)
% % % % % % % % % % % % BANDA_MORTA_PSI = 2.0;
% % % % % % % % % % % % 
% % % % % % % % % % % % %% 2. MEMÓRIA INTERNA DA ECU
% % % % % % % % % % % % persistent z_est erro_int_acum
% % % % % % % % % % % % if isempty(z_est)
% % % % % % % % % % % %     z_est         = [0.0; 0.0; 0.0]; 
% % % % % % % % % % % %     erro_int_acum = 0.0;             
% % % % % % % % % % % % end
% % % % % % % % % % % % 
% % % % % % % % % % % % %% 3. LEITURA DOS SENSORES E CÁLCULO DO ERRO
% % % % % % % % % % % % P_roda_pa = double(P_roda_psi) * PSI_TO_PA;
% % % % % % % % % % % % P_ref_pa  = double(P_ref_psi) * PSI_TO_PA;
% % % % % % % % % % % % erro_psi  = double(P_ref_psi) - double(P_roda_psi);
% % % % % % % % % % % % 
% % % % % % % % % % % % %% 4. OBSERVADOR DE LUENBERGER (Sempre atualizando o estado do motor)
% % % % % % % % % % % % y_est = C * z_est;
% % % % % % % % % % % % erro_estimacao = P_roda_pa - y_est;
% % % % % % % % % % % % z_dot_est = A * z_est + B * (double(erro_int_acum) * K_i - K_est * z_est) + L * erro_estimacao;
% % % % % % % % % % % % z_est     = z_est + z_dot_est * dt;
% % % % % % % % % % % % 
% % % % % % % % % % % % %% 5. GERENCIADOR LÓGICO DE FASE (APPLY, HOLD, RELEASE)
% % % % % % % % % % % % 
% % % % % % % % % % % % if erro_psi > BANDA_MORTA_PSI
% % % % % % % % % % % %     %% --- FASE DE AUMENTO (APPLY) ---
% % % % % % % % % % % %     % Precisa de pressão: abre as vias do LAC para a roda
% % % % % % % % % % % %     u_mcv = 0; % Isolado do reservatório
% % % % % % % % % % % %     u_pfv = 1; % LAC alimenta a linha principal
% % % % % % % % % % % %     u_irl = 1; % Linha principal alimenta a roda
% % % % % % % % % % % %     u_orl = 0; % Exaustão fechada
% % % % % % % % % % % % 
% % % % % % % % % % % %     % Integra o erro e calcula a ação do LQI para empurrar o motor
% % % % % % % % % % % %     erro_pressao  = P_ref_pa - P_roda_pa;
% % % % % % % % % % % %     erro_int_acum = erro_int_acum + erro_pressao * dt;
% % % % % % % % % % % %     u_controle    = - (K_est * z_est) + (K_i * erro_int_acum);
% % % % % % % % % % % %     duty_cycle_ecu = u_controle * 100;
% % % % % % % % % % % % 
% % % % % % % % % % % % elseif erro_psi < -BANDA_MORTA_PSI
% % % % % % % % % % % %     %% --- FASE DE ALÍVIO (RELEASE / DUMP) ---
% % % % % % % % % % % %     % Sobrou pressão: abre a exaustão da roda para o reservatório
% % % % % % % % % % % %     u_mcv = 0;
% % % % % % % % % % % %     u_pfv = 0;
% % % % % % % % % % % %     u_irl = 0; % Isola a linha principal para reter o nó 1
% % % % % % % % % % % %     u_orl = 1; % Abre exaustão da roda direto para o reservatório
% % % % % % % % % % % % 
% % % % % % % % % % % %     % Reseta o integrador do LQI para evitar o estouro de ganho (Anti-windup)
% % % % % % % % % % % %     erro_int_acum = 0.0;
% % % % % % % % % % % % 
% % % % % % % % % % % %     % Comanda o motor do LAC para recuar de forma controlada para a parede inicial
% % % % % % % % % % % %     duty_cycle_ecu = -30.0; % Recuo fixo de segurança (30% PWM invertido)
% % % % % % % % % % % % 
% % % % % % % % % % % % else
% % % % % % % % % % % %     %% --- FASE DE RETENÇÃO (HOLD) ---
% % % % % % % % % % % %     % A pressão atingiu o alvo dentro da banda estável: sela o caliper
% % % % % % % % % % % %     u_mcv = 0;
% % % % % % % % % % % %     u_pfv = 0;
% % % % % % % % % % % %     u_irl = 0; % FECHA A IRL: Aprisiona o óleo dentro do caliper da roda
% % % % % % % % % % % %     u_orl = 0;
% % % % % % % % % % % % 
% % % % % % % % % % % %     % Congela o integrador para manter a memória do último esforço
% % % % % % % % % % % %     u_controle    = - (K_est * z_est) + (K_i * erro_int_acum);
% % % % % % % % % % % %     duty_cycle_ecu = u_controle * 100;
% % % % % % % % % % % % 
% % % % % % % % % % % %     % Como as válvulas travaram a pressão mecanicamente, podemos desligar o motor
% % % % % % % % % % % %     duty_cycle_ecu = 0.0; 
% % % % % % % % % % % % end
% % % % % % % % % % % % 
% % % % % % % % % % % % %% 6. SATURAÇÃO DE SEGURANÇA DO MOTOR
% % % % % % % % % % % % if duty_cycle_ecu > 100.0
% % % % % % % % % % % %     duty_cycle_ecu = 100.0;
% % % % % % % % % % % % elseif duty_cycle_ecu < -100.0
% % % % % % % % % % % %     duty_cycle_ecu = -100.0;
% % % % % % % % % % % % end
% % % % % % % % % % % % 
% % % % % % % % % % % % end
% % % % % % % % % % % % 
% % % % % % % % % % % % % function duty_cycle_ecu = ecu_control_fcn(P_roda_psi, P_ref_psi, dt)
% % % % % % % % % % % % % %#codegen
% % % % % % % % % % % % % % ALGORITMO EMBARCADO DA ECU: CONTROLADOR LQI + OBSERVADOR DE LUENBERGER
% % % % % % % % % % % % % % Inputs:
% % % % % % % % % % % % % %   P_roda_psi   : Sinal lido do sensor físico da roda [PSI]
% % % % % % % % % % % % % %   P_ref_psi    : Referência de pressão desejada [PSI]
% % % % % % % % % % % % % %   dt           : Passo de tempo da malha de controle (ex: 0.001 s)
% % % % % % % % % % % % % % Output:
% % % % % % % % % % % % % %   duty_cycle_ecu : Sinal de PWM enviado para o motor (-100 a 100)
% % % % % % % % % % % % % 
% % % % % % % % % % % % % %% 1. VETORES DE GANHO (Cole aqui os valores numéricos gerados pelo Script do Passo 1)
% % % % % % % % % % % % % % Exemplo de valores pré-calculados de referência:
% % % % % % % % % % % % % K_est = [3.1623,   0.0242,   0.000302];  % Ganhos de [x, x_dot, P_pa]
% % % % % % % % % % % % % K_i   = -22.3607;                        % Ganho do integrador
% % % % % % % % % % % % % 
% % % % % % % % % % % % % L = [21.41; 1654.21; 42.85];             % Ganhos do Observador de Luenberger
% % % % % % % % % % % % % 
% % % % % % % % % % % % % % Constantes físicas fixas para conversão internas da ECU
% % % % % % % % % % % % % PSI_TO_PA = 6894.757;
% % % % % % % % % % % % % A_lac     = 2.85e-4;
% % % % % % % % % % % % % tau_m     = 0.140;
% % % % % % % % % % % % % K_drv     = 0.085;
% % % % % % % % % % % % % C_eq      = 9.51e-12; % Capacitância equivalente calculada pelo script
% % % % % % % % % % % % % 
% % % % % % % % % % % % % % Matrizes de Espaço de Estados do Modelo Interno da ECU
% % % % % % % % % % % % % A = [0,       1,       0;
% % % % % % % % % % % % %      0,  -1/tau_m,     0;
% % % % % % % % % % % % %      0, A_lac/C_eq,    0];
% % % % % % % % % % % % % 
% % % % % % % % % % % % % B = [0; K_drv/tau_m; 0];
% % % % % % % % % % % % % C = [0, 0, 1];
% % % % % % % % % % % % % 
% % % % % % % % % % % % % %% 2. DECLARAÇÃO DOS ESTADOS INTERNOS (MEMÓRIA DA ECU)
% % % % % % % % % % % % % persistent z_est erro_int_acum
% % % % % % % % % % % % % 
% % % % % % % % % % % % % if isempty(z_est)
% % % % % % % % % % % % %     z_est          = [0.0; 0.0; 0.0]; % Estados estimados iniciais: [x_est; x_dot_est; p_est]
% % % % % % % % % % % % %     erro_int_acum  = 0.0;             % Acumulador da ação integral
% % % % % % % % % % % % % end
% % % % % % % % % % % % % 
% % % % % % % % % % % % % %% 3. CONVERSÃO DE UNIDADES DO MUNDO REAL PARA O SISTEMA INTERNACIONAL (SI)
% % % % % % % % % % % % % P_roda_pa = double(P_roda_psi) * PSI_TO_PA;
% % % % % % % % % % % % % P_ref_pa  = double(P_ref_psi) * PSI_TO_PA;
% % % % % % % % % % % % % 
% % % % % % % % % % % % % %% 4. ALGORITMO DO OBSERVADOR DE LUENBERGER (Estimação de x e x_dot sem sensores)
% % % % % % % % % % % % % % Cálculo do erro de estimação da saída (Y_real - Y_estimado)
% % % % % % % % % % % % % y_est = C * z_est;
% % % % % % % % % % % % % erro_estimacao = P_roda_pa - y_est;
% % % % % % % % % % % % % 
% % % % % % % % % % % % % % Equação dinâmica do observador de Luenberger (Discretizado via Euler)
% % % % % % % % % % % % % z_dot_est = A * z_est + B * (double(erro_int_acum) * K_i - K_est * z_est) + L * erro_estimacao;
% % % % % % % % % % % % % z_est     = z_est + z_dot_est * dt;
% % % % % % % % % % % % % 
% % % % % % % % % % % % % %% 5. CÁLCULO DA AÇÃO INTEGRAL DO LQI
% % % % % % % % % % % % % % Erro atual de rastreamento de pressão
% % % % % % % % % % % % % erro_pressao = P_ref_pa - P_roda_pa;
% % % % % % % % % % % % % 
% % % % % % % % % % % % % % Integração numérica do erro para eliminar erro em regime permanente
% % % % % % % % % % % % % erro_int_acum = erro_int_acum + erro_pressao * dt;
% % % % % % % % % % % % % 
% % % % % % % % % % % % % %% 6. LEI DE CONTROLE LQI (Cálculo do esforço de controle u)
% % % % % % % % % % % % % % u = -K*z_est + Ki*erro_int
% % % % % % % % % % % % % u_controle = - (K_est * z_est) + (K_i * erro_int_acum);
% % % % % % % % % % % % % 
% % % % % % % % % % % % % %% 7. SATURAÇÃO E MAPEAMENTO DO SINAL DE PWM DA ECU
% % % % % % % % % % % % % % O comando 'u_controle' sai em fração (0 a 1). Convertemos para escala de PWM da bancada (-100 a 100%)
% % % % % % % % % % % % % duty_cycle_ecu = u_controle * 100;
% % % % % % % % % % % % % 
% % % % % % % % % % % % % % Limitação física de segurança eletrônica da ponte H do motor
% % % % % % % % % % % % % if duty_cycle_ecu > 100.0
% % % % % % % % % % % % %     duty_cycle_ecu = 100.0;
% % % % % % % % % % % % % elseif duty_cycle_ecu < -100.0
% % % % % % % % % % % % %     duty_cycle_ecu = -100.0;
% % % % % % % % % % % % % end
% % % % % % % % % % % % % 
% % % % % % % % % % % % % end
